simulink model "PMSMPlantTest"  (R2026b)
settings: Solver=ode4  StopTime=fixtureCfg.Duration  FixedStep=experimentCfg.Step
PostLoadFcn:
  | addpath(fullfile(fileparts(fileparts(fileparts(fileparts(fileparts(get_param(bdroot,'FileName')))))),'docs','scripts'));initialize_motor_paths();initialize_motor_model(bdroot);
model workspace (MAT data in the model file):
  currentCfg.Ts = 0.0001
  currentCfg.BandwidthHz = 500
  currentCfg.Kpd = 3.14159265359
  currentCfg.Kpq = 3.76991118431
  currentCfg.Kid = 1570.79632679
  currentCfg.Kiq = 1570.79632679
  currentCfg.Kaw = 1000
  deadtimeCfg.DeadTime = 2e-06
  deadtimeCfg.DeviceDrop = 0
  deadtimeCfg.CurrentBlend = 0.1
  deadtimeCfg.ModelEnable = 0
  deadtimeCfg.CompensationEnable = 0
  deadtimeCfg.CompensationScale = 1
  deadtimeCfg.SwitchingStep = 1e-07
  experimentCfg.Step = 5e-06
  experimentCfg.LogTs = 0.0001
  experimentCfg.Duration = 1.5
  experimentCfg.Mode = 2
  experimentCfg.UseInverter = 1
  experimentCfg.UseTiming = 1
  experimentCfg.UseMechanical = 1
  experimentCfg.ImposedElectricalSpeed = 0
  experimentCfg.IdReference = 0
  experimentCfg.IqReference = 2
  experimentCfg.IqInitial = 0
  experimentCfg.SpeedReference = 40
  experimentCfg.SpeedInitial = 0
  experimentCfg.PositionReference = 1
  experimentCfg.PositionInitial = 0
  experimentCfg.CommandTime = 0.05
  experimentCfg.LoadTorque = 0.1
  experimentCfg.LoadTime = 0.35
  experimentCfg.Enable = 1
  experimentCfg.Reset = 0
  feedforwardCfg.Enable = 0
  feedforwardCfg.ParameterScale = 1
  fixtureCfg.Ts = 0.0001
  fixtureCfg.Duration = 0.03
  fixtureCfg.SolverStep = 5e-06
  fixtureCfg.Vd = 2
  fixtureCfg.Vq = 0
  fixtureCfg.ElectricalSpeed = 0
  fixtureCfg.MechanicalTorque = 0
  fixtureCfg.LoadTorque = 0
  fixtureCfg.Inputs = [2 2 2 2 2 2 2 2 2 2 2 2 ... (1505 elements, 301x5)]
  inverterCfg.Vdc = 48
  inverterCfg.MinDuty = 0.02
  inverterCfg.PwmTs = 0.0001
  inverterCfg.LinearLimit = 26.6043004043
  motionCfg.Ts = 0.001
  motionCfg.NaturalFrequency = 20
  motionCfg.Damping = 0.9
  motionCfg.Kt = 0.21
  motionCfg.Kp = 0.0852380952381
  motionCfg.Ki = 0.952380952381
  motionCfg.Kaw = 20
  motionCfg.PositionKp = 8
  motionCfg.SpeedLimit = 80
  motionCfg.AccelerationLimit = 200
  motionCfg.CurrentLimit = 8
  pmsmCfg.Rs = 0.5
  pmsmCfg.Ld = 0.001
  pmsmCfg.Lq = 0.0012
  pmsmCfg.Flux = 0.035
  pmsmCfg.PolePairs = 4
  pmsmCfg.J = 0.0005
  pmsmCfg.B = 0.0001
  pmsmCfg.Id0 = 0
  pmsmCfg.Iq0 = 0
  pmsmCfg.Speed0 = 0
  pmsmCfg.Position0 = 0
  testStim.time = []
  testStim.signals.values = [2 2 2 2 2 2 2 2 2 2 2 2 ... (1505 elements, 301x5)]
  testStim.signals.dimensions = 5
  timingCfg.Ts = 0.0001
  timingCfg.FeedbackTicks = 1
  timingCfg.ActuationTicks = 1
libraries: PMSMPlant x2
settings Model: Creator=24322  LastModifiedBy=24322

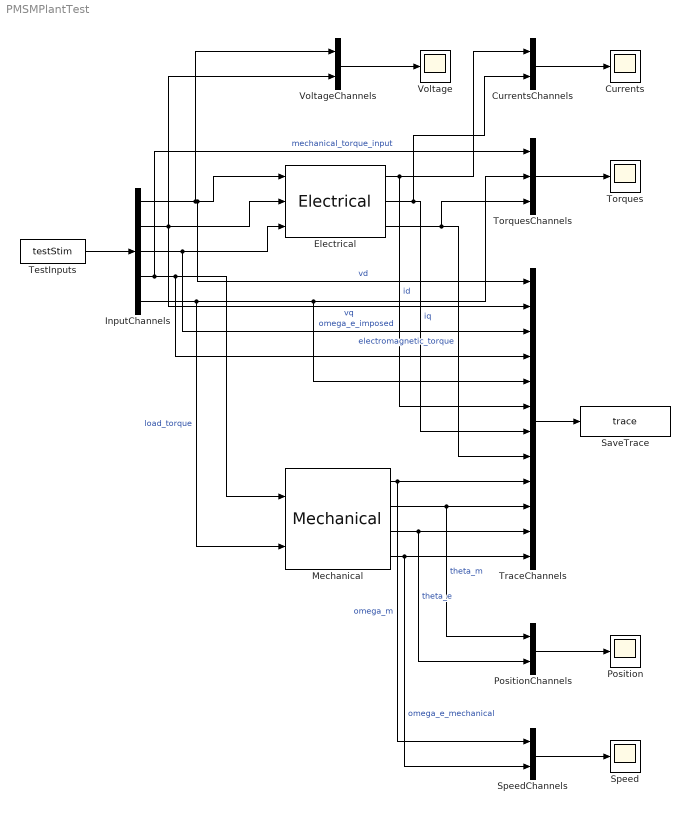
== system PMSMPlantTest ==
  Currents : Scope
      settings: Title=Currents  YLabel=A
  CurrentsChannels : Mux  Inputs=2
  Electrical : PMSMPlant/Electrical  SystemSampleTime=-1  VariantActivationTime=update diagram  EmptyChoice=off  PassThrough=off  PassThroughVariantControl=(default)  EmptyChoiceVariantControl=(default)  AllowFlexibleInterface=on  Latency=0  AutoFrameSizeCalculation=off
  InputChannels : Demux  Outputs=5
  Mechanical : PMSMPlant/Mechanical  SystemSampleTime=-1  VariantActivationTime=update diagram  EmptyChoice=off  PassThrough=off  PassThroughVariantControl=(default)  EmptyChoiceVariantControl=(default)  AllowFlexibleInterface=on  Latency=0  AutoFrameSizeCalculation=off
  Position : Scope
      settings: Title=Position  YLabel=rad
  PositionChannels : Mux  Inputs=2
  SaveTrace : ToWorkspace  VariableName=trace  SaveFormat=Structure With Time  SampleTime=experimentCfg.LogTs
  Speed : Scope
      settings: Title=Speed  YLabel=rad/s
  SpeedChannels : Mux  Inputs=2
  TestInputs : FromWorkspace  VariableName=testStim  SampleTime=currentCfg.Ts  Interpolate=off  OutputAfterFinalValue=Holding final value
  Torques : Scope
      settings: Title=Torques  YLabel=N*m
  TorquesChannels : Mux  Inputs=3
  TraceChannels : Mux  Inputs=12
  Voltage : Scope
      settings: Title=Voltage  YLabel=V
  VoltageChannels : Mux  Inputs=2
  wires:
  VoltageChannels/1 -> Voltage/1
  PositionChannels/1 -> Position/1
  SpeedChannels/1 -> Speed/1
  TorquesChannels/1 -> Torques/1
  CurrentsChannels/1 -> Currents/1
  Mechanical/4 -> TraceChannels/12, SpeedChannels/2  "omega_e_mechanical"
  Mechanical/3 -> TraceChannels/11, PositionChannels/2  "theta_e"
  Mechanical/2 -> TraceChannels/10, PositionChannels/1  "theta_m"
  Mechanical/1 -> TraceChannels/9, SpeedChannels/1  "omega_m"
  Electrical/3 -> TraceChannels/8, TorquesChannels/3  "electromagnetic_torque"
  Electrical/2 -> TraceChannels/7, CurrentsChannels/2  "iq"
  Electrical/1 -> TraceChannels/6, CurrentsChannels/1  "id"
  TraceChannels/1 -> SaveTrace/1
  InputChannels/5 -> TraceChannels/5, TorquesChannels/2, Mechanical/2  "load_torque"
  InputChannels/4 -> TraceChannels/4, Mechanical/1, TorquesChannels/1  "mechanical_torque_input"
  InputChannels/3 -> Electrical/3, TraceChannels/3  "omega_e_imposed"
  InputChannels/2 -> VoltageChannels/2, Electrical/2, TraceChannels/2  "vq"
  InputChannels/1 -> TraceChannels/1, Electrical/1, VoltageChannels/1  "vd"
  TestInputs/1 -> InputChannels/1
